simulink model "PMLSM_ControlCore_Block"  (R2026a)
settings: Solver=FixedStepDiscrete  StopTime=1  FixedStep=1e-4
values from neighbouring files (symbols this model uses):
  CPU_Clock = 200e6    (= 200000000)    [PMSLM_Init_Params_MBDL4.m]
  Current_Control_Mode = 2    [init_PMLSM_mil_test_params.m]
  DeadTime_Comp_Enable = 0    [init_PMLSM_mil_test_params.m]
  delay_N = 50    [PMSLM_Init_Params_MBDL4.m]
  DPCC_Ld_Factor = 1    [init_PMLSM_mil_test_params.m]
  DPCC_Lq_Factor = 1    [init_PMLSM_mil_test_params.m]
  DPCC_Psi_Factor = 1    [init_PMLSM_mil_test_params.m]
  DPCC_Rs_Factor = 1    [init_PMLSM_mil_test_params.m]
  DPICC_Ld_Factor = 1    [init_PMLSM_mil_test_params.m]
  DPICC_Lq_Factor = 1    [init_PMLSM_mil_test_params.m]
  Hold_Ticks = 30000    [PMSLM_Init_Params_MBDL4.m]
  Id_Init_Step = Id_Init_Target / Ramp_Ticks    (= 5e-05)    [PMSLM_Init_Params_MBDL4.m]
  Id_Init_Target = 0.5    [PMSLM_Init_Params_MBDL4.m]
  Id_Release_Ramp_Ticks = 2000    [PMSLM_Init_Params_MBDL4.m]
  Iq_fric_run = 0.05    [PMSLM_Init_Params_MBDL4.m]
  Iq_fric_start = 0.40    (= 0.4)    [PMSLM_Init_Params_MBDL4.m]
  Iq_int_limit = 0.10    (= 0.1)    [PMSLM_Init_Params_MBDL4.m]
  Kaw_d = Kaw_q    (= 0.2)    [PMSLM_Init_Params_MBDL4.m]
  Kaw_q = 0.2    [PMSLM_Init_Params_MBDL4.m]
  Kaw_s = 0.4    [PMSLM_Init_Params_MBDL4.m]
  Ki_ACR = ACR_Commissioning_Scale*Ki_ACR_Baseline    (= 2962.5)    [PMSLM_Init_Params_MBDL4.m]    (also in init_PMLSM_mil_test_params.m = Kp_ACR*PMLSM_Rs_ohm/PMLSM_Lq_H)
  Ki_ASR = 0.05    [PMSLM_Init_Params_MBDL4.m]
  Kp_ACR = ACR_Commissioning_Scale*Kp_ACR_Baseline    (= 2.18125)    [PMSLM_Init_Params_MBDL4.m]    (also in init_PMLSM_mil_test_params.m = PMLSM_Lq_H/(4*MIL_AUM3S4_Current_PI_xi^2*MIL_AUM3S4_Current_)
  Kp_ASR = 0.03    [PMSLM_Init_Params_MBDL4.m]
  Kp_pos = 5    [PMSLM_Init_Params_MBDL4.m]
  PICDO_Dhat_Limit_A = 3.0    (= 3)    [init_PMLSM_mil_test_params.m]
  PICDO_Kd = 0.25    [init_PMLSM_mil_test_params.m]
  PICDO_Kx = 1.0    (= 1)    [init_PMLSM_mil_test_params.m]
  PMLSM_deadtime_ratio = PMLSM_deadtime_s * PMLSM_pwm_freq_Hz    (= 0.01)    [init_PMLSM_plant_params.m]
  PMLSM_Ld_H = Ld    (= 0.001745)    [PMSLM_Init_Params_MBDL4.m]    (also in init_PMLSM_plant_params.m)
  PMLSM_Lq_H = Lq    (= 0.001745)    [PMSLM_Init_Params_MBDL4.m]    (also in init_PMLSM_plant_params.m)
  PMLSM_psi_f_Wb = flux    (= 0.141)    [PMSLM_Init_Params_MBDL4.m]    (also in init_PMLSM_plant_params.m)
  PMLSM_Rs_ohm = Rs    (= 2.37)    [PMSLM_Init_Params_MBDL4.m]    (also in init_PMLSM_plant_params.m)
  Pos_deadband = 0.02    [PMSLM_Init_Params_MBDL4.m]
  Ramp_Ticks = 10000    [PMSLM_Init_Params_MBDL4.m]
  Speed_Feedback_Mode = 1    [init_PMLSM_mil_test_params.m]
  Speed_loop_Iq_Limit = Iq_Limit    (= 0.3)    [PMSLM_Init_Params_MBDL4.m]
  Tau_e_mm = 60    [PMSLM_Init_Params_MBDL4.m]
  theta_align_const = 0    [PMSLM_Init_Params_MBDL4.m]
  Theta_Offset_Fine = Simulink.Parameter    [PMSLM_Init_Params_MBDL4.m]
  Ts = 1 / PWM_Freq    (= 0.0001)    [PMSLM_Init_Params_MBDL4.m]
  Ts_ACR = 1e-4    (= 0.0001)    [PMSLM_Init_Params_MBDL4.m]
  Ts_ASR = 1e-3    (= 0.001)    [PMSLM_Init_Params_MBDL4.m]
  Ts_DPICC = 1e-4    (= 0.0001)    [init_PMLSM_mil_test_params.m]
  Udc = 48    [PMSLM_Init_Params_MBDL4.m]    (also in init_PMLSM_mil_test_params.m)
  Uq_Zero_EN = 0：q 轴用正常 PI    [PMSLM_Init_Params_MBDL4.m]
  v_ff_eps = 0.5    [PMSLM_Init_Params_MBDL4.m]
  V_meas_max = 500    [PMSLM_Init_Params_MBDL4.m]
  v_meas_zero_eps = 0.5    [PMSLM_Init_Params_MBDL4.m]
  v_over_eps = 3    [PMSLM_Init_Params_MBDL4.m]
  V_pos_max_mmps = 10    [PMSLM_Init_Params_MBDL4.m]
  v_ref_max = 20    [PMSLM_Init_Params_MBDL4.m]
  v_ref_set_step_dn = v_ref_set_rate_dn * Ts    (= 0.005)    [PMSLM_Init_Params_MBDL4.m]
  v_ref_set_step_up = v_ref_set_rate_up * Ts    (= 0.005)    [PMSLM_Init_Params_MBDL4.m]
  v_ref_zero_eps = 0.2    [PMSLM_Init_Params_MBDL4.m]
  v_stick_off = 3.0    (= 3)    [PMSLM_Init_Params_MBDL4.m]
  v_stick_on = 1.0    (= 1)    [PMSLM_Init_Params_MBDL4.m]
  X_max_hard = 500    [PMSLM_Init_Params_MBDL4.m]
  X_max_soft = 470    [PMSLM_Init_Params_MBDL4.m]
  X_min_hard = -500    [PMSLM_Init_Params_MBDL4.m]
  X_min_soft = -470    [PMSLM_Init_Params_MBDL4.m]
libraries: hdlsllib x13, simulink x11, mcbeeMathTransformLib x2, mcbcontrolslib x1
(part 1 of 3)
settings Model: Creator=lww  LastModifiedBy=lww
settings ModelReferenceCC: ModelReferenceNumInstancesAllowed=Single
settings GRTTargetCC: SubcomponentCodeInterfacePackaging=Nonreusable function

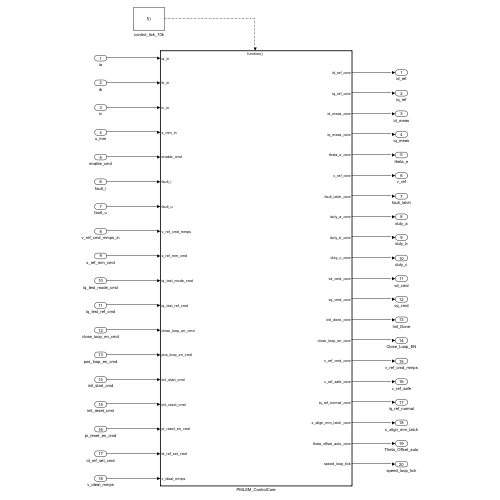
[thumbnail: Simulink's stored preview of the top-level diagram]
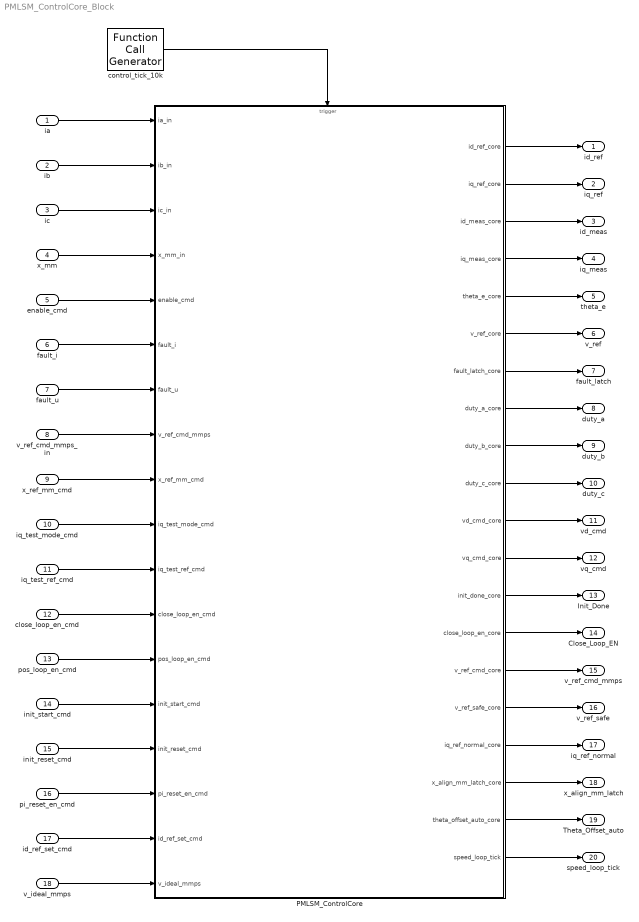
== system PMLSM_ControlCore_Block ==
  ia : Inport
  ib : Inport  Port=2
  ic : Inport  Port=3
  x_mm : Inport  Port=4
  enable_cmd : Inport  Port=5
  fault_i : Inport  Port=6
  fault_u : Inport  Port=7
  v_ref_cmd_mmps_in : Inport  Port=8
  x_ref_mm_cmd : Inport  Port=9
  iq_test_mode_cmd : Inport  Port=10
  iq_test_ref_cmd : Inport  Port=11
  close_loop_en_cmd : Inport  Port=12
  pos_loop_en_cmd : Inport  Port=13
  init_start_cmd : Inport  Port=14
  init_reset_cmd : Inport  Port=15
  pi_reset_en_cmd : Inport  Port=16
  id_ref_set_cmd : Inport  Port=17
  v_ideal_mmps : Inport  Port=18
  PMLSM_ControlCore : Subsystem  TreatAsAtomicUnit=on
  control_tick_10k : FunctionCallGenerator  SampleTime=1e-4
  id_ref : Outport
  iq_ref : Outport  Port=2
  id_meas : Outport  Port=3
  iq_meas : Outport  Port=4
  theta_e : Outport  Port=5
  v_ref : Outport  Port=6
  fault_latch : Outport  Port=7
  duty_a : Outport  Port=8
  duty_b : Outport  Port=9
  duty_c : Outport  Port=10
  vd_cmd : Outport  Port=11
  vq_cmd : Outport  Port=12
  Init_Done : Outport  Port=13
  Close_Loop_EN : Outport  Port=14
  v_ref_cmd_mmps : Outport  Port=15
  v_ref_safe : Outport  Port=16
  iq_ref_normal : Outport  Port=17
  x_align_mm_latch : Outport  Port=18
  Theta_Offset_auto : Outport  Port=19
  speed_loop_tick : Outport  Port=20
  wires:
  ia/1 -> PMLSM_ControlCore/1(ia_in)
  ib/1 -> PMLSM_ControlCore/2(ib_in)
  ic/1 -> PMLSM_ControlCore/3(ic_in)
  x_mm/1 -> PMLSM_ControlCore/4(x_mm_in)
  enable_cmd/1 -> PMLSM_ControlCore/5(enable_cmd)
  fault_i/1 -> PMLSM_ControlCore/6(fault_i)
  fault_u/1 -> PMLSM_ControlCore/7(fault_u)
  v_ref_cmd_mmps_in/1 -> PMLSM_ControlCore/8(v_ref_cmd_mmps)
  x_ref_mm_cmd/1 -> PMLSM_ControlCore/9(x_ref_mm_cmd)
  iq_test_mode_cmd/1 -> PMLSM_ControlCore/10(iq_test_mode_cmd)
  iq_test_ref_cmd/1 -> PMLSM_ControlCore/11(iq_test_ref_cmd)
  close_loop_en_cmd/1 -> PMLSM_ControlCore/12(close_loop_en_cmd)
  pos_loop_en_cmd/1 -> PMLSM_ControlCore/13(pos_loop_en_cmd)
  init_start_cmd/1 -> PMLSM_ControlCore/14(init_start_cmd)
  init_reset_cmd/1 -> PMLSM_ControlCore/15(init_reset_cmd)
  pi_reset_en_cmd/1 -> PMLSM_ControlCore/16(pi_reset_en_cmd)
  id_ref_set_cmd/1 -> PMLSM_ControlCore/17(id_ref_set_cmd)
  control_tick_10k/1 -> PMLSM_ControlCore/Trigger
  PMLSM_ControlCore/1(id_ref_core) -> id_ref/1
  PMLSM_ControlCore/2(iq_ref_core) -> iq_ref/1
  PMLSM_ControlCore/3(id_meas_core) -> id_meas/1
  PMLSM_ControlCore/4(iq_meas_core) -> iq_meas/1
  PMLSM_ControlCore/5(theta_e_core) -> theta_e/1
  PMLSM_ControlCore/6(v_ref_core) -> v_ref/1
  PMLSM_ControlCore/7(fault_latch_core) -> fault_latch/1
  PMLSM_ControlCore/8(duty_a_core) -> duty_a/1
  PMLSM_ControlCore/9(duty_b_core) -> duty_b/1
  PMLSM_ControlCore/10(duty_c_core) -> duty_c/1
  PMLSM_ControlCore/11(vd_cmd_core) -> vd_cmd/1
  PMLSM_ControlCore/12(vq_cmd_core) -> vq_cmd/1
  PMLSM_ControlCore/13(init_done_core) -> Init_Done/1
  PMLSM_ControlCore/14(close_loop_en_core) -> Close_Loop_EN/1
  PMLSM_ControlCore/15(v_ref_cmd_core) -> v_ref_cmd_mmps/1
  PMLSM_ControlCore/16(v_ref_safe_core) -> v_ref_safe/1
  PMLSM_ControlCore/17(iq_ref_normal_core) -> iq_ref_normal/1
  PMLSM_ControlCore/18(x_align_mm_latch_core) -> x_align_mm_latch/1
  PMLSM_ControlCore/19(theta_offset_auto_core) -> Theta_Offset_auto/1
  v_ideal_mmps/1 -> PMLSM_ControlCore/18(v_ideal_mmps)
  PMLSM_ControlCore/20(speed_loop_tick) -> speed_loop_tick/1

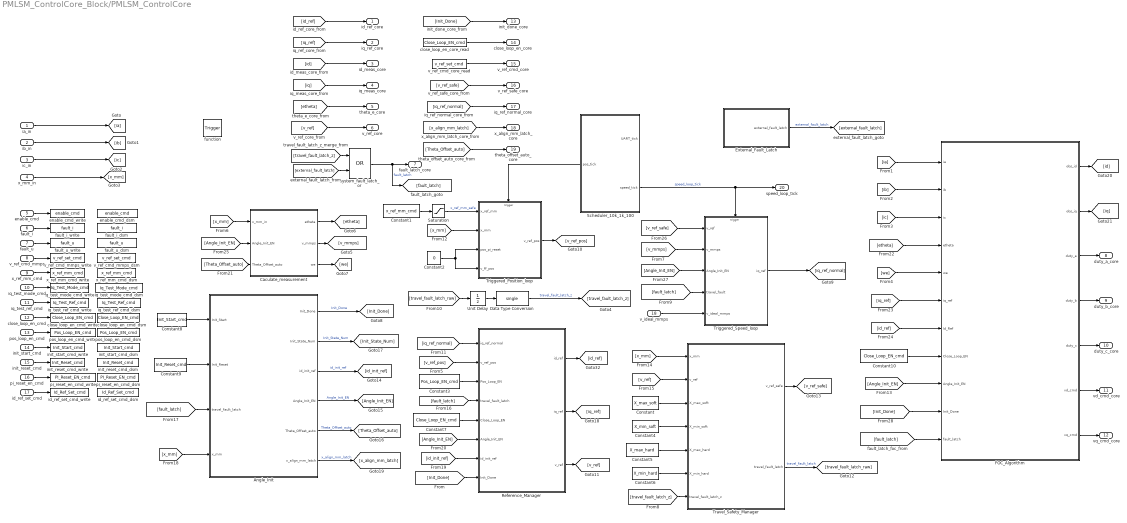
== system PMLSM_ControlCore_Block/PMLSM_ControlCore ==
  ia_in : Inport
  ib_in : Inport  Port=2
  ic_in : Inport  Port=3
  x_mm_in : Inport  Port=4
  enable_cmd : Inport  Port=5
  fault_i : Inport  Port=6
  fault_u : Inport  Port=7
  v_ref_cmd_mmps : Inport  Port=8
  x_ref_mm_cmd : Inport  Port=9
  iq_test_mode_cmd : Inport  Port=10
  iq_test_ref_cmd : Inport  Port=11
  close_loop_en_cmd : Inport  Port=12
  pos_loop_en_cmd : Inport  Port=13
  init_start_cmd : Inport  Port=14
  init_reset_cmd : Inport  Port=15
  pi_reset_en_cmd : Inport  Port=16
  id_ref_set_cmd : Inport  Port=17
  v_ideal_mmps : Inport  Port=18
  function : TriggerPort  TriggerType=function-call  VariantControl=(inherit)
  Angle_Init : Stateflow chart  TreatAsAtomicUnit=on
  Caculate_measurement : Subsystem
  Constant : Constant  Value=X_max_soft
  Constant1 : DataStoreRead  DataStoreName=x_ref_mm_cmd  IndexOptions=Index vector (dialog)  Indices=1  OutputSizes=1
  Constant10 : DataStoreRead  DataStoreName=Close_Loop_EN_cmd  IndexOptions=Index vector (dialog)  Indices=1  OutputSizes=1
  Constant2 : Constant  Value=0
  Constant3 : DataStoreRead  DataStoreName=Pos_Loop_EN_cmd  IndexOptions=Index vector (dialog)  Indices=1  OutputSizes=1
  Constant4 : Constant  Value=X_min_soft
  Constant5 : Constant  Value=X_max_hard
  Constant6 : Constant  Value=X_min_hard
  Constant7 : DataStoreRead  DataStoreName=Close_Loop_EN_cmd  IndexOptions=Index vector (dialog)  Indices=1  OutputSizes=1
  Constant8 : DataStoreRead  DataStoreName=Init_Start_cmd  IndexOptions=Index vector (dialog)  Indices=1  OutputSizes=1
  Constant9 : DataStoreRead  DataStoreName=Init_Reset_cmd  IndexOptions=Index vector (dialog)  Indices=1  OutputSizes=1
  Data Type Conversion : DataTypeConversion  OutDataTypeStr=single  SaturateOnIntegerOverflow=off  RndMeth=Floor
  External_Fault_Latch : Subsystem
  FOC_Algorithm : Subsystem
  Reference_Manager : Subsystem
  Saturation : Saturate  UpperLimit=X_max_soft  LowerLimit=X_min_soft
  Scheduler_10k_1k_100 : Subsystem
      settings: PortSchema="{\"entries\":[{\"content\":{\"sides\":[{\"content\":{\"connectorIds\":[\"Out3\"]},\"type\":\"ConnectorPlacement.EquallySpacedRectSide\",\"uuid\":\"7a2cd2ad-1b6d-4ced-b4c0-dea2e76e4441\"},{\"content\":{\"connectorIds\":[\"Out1\",\"Out2\"],\"side\":\"RIGHT\"},\"type\":\"ConnectorPlacement.EquallySpacedRectSide\",\"uuid\":\"f7db3b94-1126-4089-83bd-8e57d20e6fd7\"},{\"content\":{\"side\":\"TOP\"},\"type\":\"ConnectorPlacement.EquallySpacedRectSide\",\"uuid\":\"9153f6b5-22af-48be-92c0-68be43f93648\"}]},\"type\":\"ConnectorPlacement.EquallySpacedConnector\",\"uuid\":\"029fb485-bddc-4cd2-9c64-7547c8dffd2b\"}],\"packageUris\":[\"http://schema.mathworks.com/mf0/Connector/R2020b\"],\"version\":\"1.0\"}"
  Travel_Safety_Manager : MATLAB Function  TreatAsAtomicUnit=on
  Triggered_Position_loop : Subsystem  TreatAsAtomicUnit=on
  Triggered_Speed_loop : Subsystem  TreatAsAtomicUnit=on
  Unit Delay : UnitDelay  SampleTime=-1
  close_loop_en_cmd_dsm : DataStoreMemory  DataStoreName=Close_Loop_EN_cmd  ShowAdditionalParam=off
  close_loop_en_cmd_write : DataStoreWrite  DataStoreName=Close_Loop_EN_cmd  IndexOptions=Index vector (dialog)  Indices=1  OutputSizes=1
  close_loop_en_core_read : DataStoreRead  DataStoreName=Close_Loop_EN_cmd  IndexOptions=Index vector (dialog)  Indices=1  OutputSizes=1
  enable_cmd_dsm : DataStoreMemory  DataStoreName=enable_cmd  ShowAdditionalParam=off
  enable_cmd_write : DataStoreWrite  DataStoreName=enable_cmd  IndexOptions=Index vector (dialog)  Indices=1  OutputSizes=1
  fault_i_dsm : DataStoreMemory  DataStoreName=fault_i  ShowAdditionalParam=off
  fault_i_write : DataStoreWrite  DataStoreName=fault_i  IndexOptions=Index vector (dialog)  Indices=1  OutputSizes=1
  fault_u_dsm : DataStoreMemory  DataStoreName=fault_u  ShowAdditionalParam=off
  fault_u_write : DataStoreWrite  DataStoreName=fault_u  IndexOptions=Index vector (dialog)  Indices=1  OutputSizes=1
  id_ref_set_cmd_dsm : DataStoreMemory  DataStoreName=Id_Ref_Set_cmd  ShowAdditionalParam=off
  id_ref_set_cmd_write : DataStoreWrite  DataStoreName=Id_Ref_Set_cmd  IndexOptions=Index vector (dialog)  Indices=1  OutputSizes=1
  init_reset_cmd_dsm : DataStoreMemory  DataStoreName=Init_Reset_cmd  ShowAdditionalParam=off
  init_reset_cmd_write : DataStoreWrite  DataStoreName=Init_Reset_cmd  IndexOptions=Index vector (dialog)  Indices=1  OutputSizes=1
  init_start_cmd_dsm : DataStoreMemory  DataStoreName=Init_Start_cmd  ShowAdditionalParam=off
  init_start_cmd_write : DataStoreWrite  DataStoreName=Init_Start_cmd  IndexOptions=Index vector (dialog)  Indices=1  OutputSizes=1
  iq_test_mode_cmd_dsm : DataStoreMemory  DataStoreName=Iq_Test_Mode_cmd  ShowAdditionalParam=off
  iq_test_mode_cmd_write : DataStoreWrite  DataStoreName=Iq_Test_Mode_cmd  IndexOptions=Index vector (dialog)  Indices=1  OutputSizes=1
  iq_test_ref_cmd_dsm : DataStoreMemory  DataStoreName=Iq_Test_Ref_cmd  ShowAdditionalParam=off
  iq_test_ref_cmd_write : DataStoreWrite  DataStoreName=Iq_Test_Ref_cmd  IndexOptions=Index vector (dialog)  Indices=1  OutputSizes=1
  pi_reset_en_cmd_dsm : DataStoreMemory  DataStoreName=PI_Reset_EN_cmd  ShowAdditionalParam=off
  pi_reset_en_cmd_write : DataStoreWrite  DataStoreName=PI_Reset_EN_cmd  IndexOptions=Index vector (dialog)  Indices=1  OutputSizes=1
  pos_loop_en_cmd_dsm : DataStoreMemory  DataStoreName=Pos_Loop_EN_cmd  ShowAdditionalParam=off
  pos_loop_en_cmd_write : DataStoreWrite  DataStoreName=Pos_Loop_EN_cmd  IndexOptions=Index vector (dialog)  Indices=1  OutputSizes=1
  system_fault_latch_or : Logic  Operator=OR  AllPortsSameDT=off  OutDataTypeStr=boolean
  v_ref_cmd_core_read : DataStoreRead  DataStoreName=v_ref_set_cmd  IndexOptions=Index vector (dialog)  Indices=1  OutputSizes=1
  v_ref_cmd_mmps_dsm : DataStoreMemory  DataStoreName=v_ref_set_cmd  ShowAdditionalParam=off
  v_ref_cmd_mmps_write : DataStoreWrite  DataStoreName=v_ref_set_cmd  IndexOptions=Index vector (dialog)  Indices=1  OutputSizes=1
  x_ref_mm_cmd_dsm : DataStoreMemory  DataStoreName=x_ref_mm_cmd  ShowAdditionalParam=off
  x_ref_mm_cmd_write : DataStoreWrite  DataStoreName=x_ref_mm_cmd  IndexOptions=Index vector (dialog)  Indices=1  OutputSizes=1
  id_ref_core : Outport
  iq_ref_core : Outport  Port=2
  id_meas_core : Outport  Port=3
  iq_meas_core : Outport  Port=4
  theta_e_core : Outport  Port=5
  v_ref_core : Outport  Port=6
  fault_latch_core : Outport  Port=7
  duty_a_core : Outport  Port=8
  duty_b_core : Outport  Port=9
  duty_c_core : Outport  Port=10
  vd_cmd_core : Outport  Port=11
  vq_cmd_core : Outport  Port=12
  init_done_core : Outport  Port=13
  close_loop_en_core : Outport  Port=14
  v_ref_cmd_core : Outport  Port=15
  v_ref_safe_core : Outport  Port=16
  iq_ref_normal_core : Outport  Port=17
  x_align_mm_latch_core : Outport  Port=18
  theta_offset_auto_core : Outport  Port=19
  speed_loop_tick : Outport  Port=20
  wires:
  Scheduler_10k_1k_100/3(pos_tick) -> Triggered_Position_loop/Trigger
  FOC_Algorithm/2(obs_iq) -> [iq]
  FOC_Algorithm/1(obs_id) -> [id]
  Angle_Init/6(x_align_mm_latch) -> [x_align_mm_latch]  "x_align_mm_latch"
  [Angle_Init_EN] -> Triggered_Speed_loop/3(Angle_Init_EN)
  Angle_Init/2(Init_State_Num) -> [Init_State_Num]  "Init_State_Num"
  [Angle_Init_EN] -> Caculate_measurement/2(Angle_Init_EN)
  [Theta_Offset_auto] -> Caculate_measurement/3(Theta_Offset_auto)
  Angle_Init/5(Theta_Offset_auto) -> [Theta_Offset_auto]  "Theta_Offset_auto"
  [Angle_Init_EN] -> Reference_Manager/6(Angle_Init_EN)
  Angle_Init/4(Angle_Init_EN) -> [Angle_Init_EN]  "Angle_Init_EN"
  [id_init_ref] -> Reference_Manager/7(id_init_ref)
  Angle_Init/3(id_init_ref) -> [id_init_ref]  "id_init_ref"
  [x_mm] -> Angle_Init/4(x_mm)
  [Init_Done] -> Reference_Manager/8(Init_Done)
  Angle_Init/1(Init_Done) -> [Init_Done]  "Init_Done"
  [fault_latch] -> Angle_Init/3(travel_fault_latch)
  [fault_latch] -> Reference_Manager/4(travel_fault_latch)
  Data Type Conversion/1 -> [travel_fault_latch_z]  "travel_fault_latch_z"
  Unit Delay/1 -> Data Type Conversion/1
  [travel_fault_latch_z] -> Travel_Safety_Manager/7(travel_fault_latch_z)
  Travel_Safety_Manager/1(v_ref_safe) -> [v_ref_safe]
  Travel_Safety_Manager/2(travel_fault_latch) -> [travel_fault_latch_raw]  "travel_fault_latch"
  Constant6/1 -> Travel_Safety_Manager/6(X_min_hard)
  Constant5/1 -> Travel_Safety_Manager/5(X_max_hard)
  Constant4/1 -> Travel_Safety_Manager/4(X_min_soft)
  Constant/1 -> Travel_Safety_Manager/3(X_max_soft)
  [v_ref] -> Travel_Safety_Manager/2(v_ref)
  [x_mm] -> Travel_Safety_Manager/1(x_mm)
  [id_ref] -> FOC_Algorithm/7(Id_Ref)
  [travel_fault_latch_raw] -> Unit Delay/1
  [fault_latch] -> Triggered_Speed_loop/4(travel_fault)
  Saturation/1 -> Triggered_Position_loop/1(x_ref_mm)  "x_ref_mm_safe"
  Reference_Manager/3(v_ref) -> [v_ref]
  [x_mm] -> Caculate_measurement/1(x_mm_in)
  Caculate_measurement/3(we) -> [we]
  [v_ref_pos] -> Reference_Manager/2(v_ref_pos)
  Triggered_Position_loop/1(v_ref_pos) -> [v_ref_pos]
  Constant2/1 -> Triggered_Position_loop/3(pos_pi_reset), Triggered_Position_loop/4(v_ff_pos)
  [x_mm] -> Triggered_Position_loop/2(x_mm)
  [iq_ref] -> FOC_Algorithm/6(iq_ref)
  [we] -> FOC_Algorithm/5(we)
  [etheta] -> FOC_Algorithm/4(etheta)
  [ic] -> FOC_Algorithm/3(ic)
  [ib] -> FOC_Algorithm/2(ib)
  [ia] -> FOC_Algorithm/1(ia)
  Triggered_Speed_loop/1(iq_ref) -> [iq_ref_normal]
  Reference_Manager/2(iq_ref) -> [iq_ref]
  [v_ref_safe] -> Triggered_Speed_loop/1(v_ref)
  Scheduler_10k_1k_100/2(speed_tick) -> speed_loop_tick/1, Triggered_Speed_loop/Trigger  "speed_loop_tick"
  Reference_Manager/1(id_ref) -> [id_ref]
  Caculate_measurement/1(etheta) -> [etheta]
  [v_mmps] -> Triggered_Speed_loop/2(v_mmps)
  Caculate_measurement/2(v_mmps) -> [v_mmps]
  [iq_ref_normal] -> Reference_Manager/1(iq_ref_normal)
  ia_in/1 -> [ia]
  ib_in/1 -> [ib]
  ic_in/1 -> [ic]
  x_mm_in/1 -> [x_mm]
  enable_cmd/1 -> enable_cmd_write/1
  fault_i/1 -> fault_i_write/1
  fault_u/1 -> fault_u_write/1
  v_ref_cmd_mmps/1 -> v_ref_cmd_mmps_write/1
  x_ref_mm_cmd/1 -> x_ref_mm_cmd_write/1
  Constant1/1 -> Saturation/1
  iq_test_mode_cmd/1 -> iq_test_mode_cmd_write/1
  iq_test_ref_cmd/1 -> iq_test_ref_cmd_write/1
  close_loop_en_cmd/1 -> close_loop_en_cmd_write/1
  Constant7/1 -> Reference_Manager/5(Close_Loop_EN)
  pos_loop_en_cmd/1 -> pos_loop_en_cmd_write/1
  Constant3/1 -> Reference_Manager/3(Pos_Loop_EN)
  init_start_cmd/1 -> init_start_cmd_write/1
  Constant8/1 -> Angle_Init/1(Init_Start)
  init_reset_cmd/1 -> init_reset_cmd_write/1
  Constant9/1 -> Angle_Init/2(Init_Reset)
  pi_reset_en_cmd/1 -> pi_reset_en_cmd_write/1
  id_ref_set_cmd/1 -> id_ref_set_cmd_write/1
  [id_ref] -> id_ref_core/1
  [iq_ref] -> iq_ref_core/1
  [id] -> id_meas_core/1
  [iq] -> iq_meas_core/1
  [etheta] -> theta_e_core/1
  [v_ref] -> v_ref_core/1
  [Init_Done] -> init_done_core/1
  close_loop_en_core_read/1 -> close_loop_en_core/1
  v_ref_cmd_core_read/1 -> v_ref_cmd_core/1
  [v_ref_safe] -> v_ref_safe_core/1
  [iq_ref_normal] -> iq_ref_normal_core/1
  [x_align_mm_latch] -> x_align_mm_latch_core/1
  [Theta_Offset_auto] -> theta_offset_auto_core/1
  [travel_fault_latch_z] -> system_fault_latch_or/1
  External_Fault_Latch/1(external_fault_latch) -> [external_fault_latch]  "external_fault_latch"
  [external_fault_latch] -> system_fault_latch_or/2
  system_fault_latch_or/1 -> fault_latch_core/1, [fault_latch]  "fault_latch"
  FOC_Algorithm/3(duty_a) -> duty_a_core/1
  FOC_Algorithm/4(duty_b) -> duty_b_core/1
  FOC_Algorithm/5(duty_c) -> duty_c_core/1
  FOC_Algorithm/6(vd_cmd) -> vd_cmd_core/1
  FOC_Algorithm/7(vq_cmd) -> vq_cmd_core/1
  v_ideal_mmps/1 -> Triggered_Speed_loop/5(v_ideal_mmps)
  [Angle_Init_EN] -> FOC_Algorithm/9(Angle_Init_EN)
  Constant10/1 -> FOC_Algorithm/8(Close_Loop_EN)
  [fault_latch] -> FOC_Algorithm/11(fault_latch)
  [Init_Done] -> FOC_Algorithm/10(Init_Done)

== system PMLSM_ControlCore_Block/PMLSM_ControlCore/Caculate_measurement ==
  x_mm_in : Inport
  Angle_Init_EN : Inport  Port=2
  Theta_Offset_auto : Inport  Port=3
  Add1 : Sum  Inputs=+-
  Add2 : Sum  Inputs=+++
  Constant : Constant  Value=0
  Constant1 : Constant  Value=0
  Constant4 : Constant  Value=2*pi
  Constant6 : Constant  Value=theta_align_const
  Data Type Conversion : DataTypeConversion  OutDataTypeStr=double  SaturateOnIntegerOverflow=off  RndMeth=Floor
  Delay : Delay  DelayLength=50
  Gain : Gain  Gain=2*pi/Tau_e_mm
  Gain1 : Gain  Gain=1/(delay_N*Ts)
  Gain2 : Gain  Gain=2*pi/Tau_e_mm
  IIR Filter : Subsystem  TreatAsAtomicUnit=on
  Math Function1 : Math  Operator=mod
  Saturation : Saturate  UpperLimit=V_meas_max  LowerLimit=-V_meas_max
  Switch : Switch  Criteria=u2 > Threshold  Threshold=0.5  SaturateOnIntegerOverflow=off  InputSameDT=off
  Switch1 : Switch  Criteria=u2 > Threshold  Threshold=0.5  SaturateOnIntegerOverflow=off  InputSameDT=off
  Switch2 : Switch  Criteria=u2 > Threshold  Threshold=0.5  SaturateOnIntegerOverflow=off  InputSameDT=off
  Theta_Offset : Constant  Value=Theta_Offset_Fine
  etheta : Outport
  v_mmps : Outport  Port=2
  we : Outport  Port=3
  wires:
  Theta_Offset_auto/1 -> Add2/2
  Theta_Offset/1 -> Add2/3
  [Angle_Init_EN] -> IIR Filter/Reset, Switch1/2
  Gain2/1 -> we/1
  Constant6/1 -> Switch2/1
  Angle_Init_EN/1 -> [Angle_Init_EN]
  Switch2/1 -> etheta/1  "obs_etheta"
  Math Function1/1 -> Switch2/3  "theta_calc"
  [Angle_Init_EN] -> Switch2/2, Switch/2
  Saturation/1 -> Switch/3
  Gain1/1 -> IIR Filter/1(In1)
  IIR Filter/1(Out1) -> Saturation/1
  Add1/1 -> Switch1/3
  Switch1/1 -> Gain1/1
  Constant1/1 -> Switch1/1
  Constant/1 -> Switch/1
  Switch/1 -> v_mmps/1, Gain2/1  "obs_v_mmps"
  Data Type Conversion/1 -> Gain/1, Add1/1, Delay/1
  Constant4/1 -> Math Function1/2
  Add2/1 -> Math Function1/1
  Gain/1 -> Add2/1
  Delay/1 -> Add1/2  "x_mm_delay"
  x_mm_in/1 -> Data Type Conversion/1

== system PMLSM_ControlCore_Block/PMLSM_ControlCore/External_Fault_Latch ==
  external_fault_latch_or : Logic  Operator=OR  AllPortsSameDT=off  OutDataTypeStr=boolean
  external_fault_latch_z : UnitDelay  SampleTime=-1
  external_fault_or : Logic  Operator=OR  AllPortsSameDT=off  OutDataTypeStr=boolean
  fault_i : DataStoreRead  DataStoreName=fault_i  IndexOptions=Index vector (dialog)  Indices=1  OutputSizes=1
  fault_i_active : simulink/Logic and Bit Operations/Compare To Constant  relop=~=  const=0  OutDataTypeStr=boolean
  fault_u : DataStoreRead  DataStoreName=fault_u  IndexOptions=Index vector (dialog)  Indices=1  OutputSizes=1
  fault_u_active : simulink/Logic and Bit Operations/Compare To Constant  relop=~=  const=0  OutDataTypeStr=boolean
  external_fault_latch : Outport
  wires:
  fault_i/1 -> fault_i_active/1
  fault_u/1 -> fault_u_active/1
  fault_i_active/1 -> external_fault_or/1
  fault_u_active/1 -> external_fault_or/2
  external_fault_or/1 -> external_fault_latch_or/1
  external_fault_latch_z/1 -> external_fault_latch_or/2
  external_fault_latch_or/1 -> external_fault_latch_z/1, external_fault_latch/1

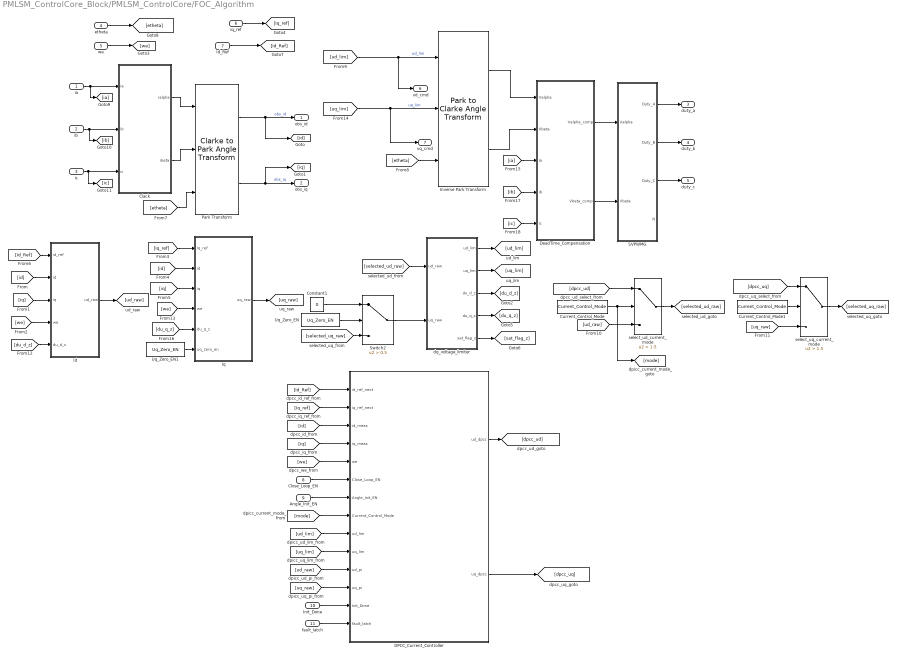
== system PMLSM_ControlCore_Block/PMLSM_ControlCore/FOC_Algorithm ==
  ia : Inport
  ib : Inport  Port=2
  ic : Inport  Port=3
  etheta : Inport  Port=4
  we : Inport  Port=5
  iq_ref : Inport  Port=6
  Id_Ref : Inport  Port=7
  Close_Loop_EN : Inport  Port=8
  Angle_Init_EN : Inport  Port=9
  Init_Done : Inport  Port=10
  fault_latch : Inport  Port=11
  Clack : Subsystem  TreatAsAtomicUnit=on  RTWFcnName=Clack_Fun
      settings: RTWFcnNameOpts=User specified
  Constant1 : Constant  Value=0  OutDataTypeStr=double
  Current_Control_Mode : Constant  Value=Current_Control_Mode
  Current_Control_Mode1 : Constant  Value=Current_Control_Mode
  DPCC_Current_Controller : Subsystem
  DeadTime_Compensation : Subsystem
  Id : Subsystem  TreatAsAtomicUnit=on  RTWFcnName=Id_Fun
      settings: RTWFcnNameOpts=User specified
  Inverse Park Transform : mcbeeMathTransformLib/Park to Clarke Angle Transform  AxisAlignment=D-axis  UseWithEmbedded=on  PhaseInput=Two inputs  ThetaInput=Electrical position  AngleInput=Radians  N_points=1024
      settings: LibrarySourceBlock=mcbhdllib/Controls/Math Transforms/Inverse Park Transform
  Iq : Subsystem  TreatAsAtomicUnit=on  RTWFcnName=Iq_Fun
      settings: RTWFcnNameOpts=User specified
  Park Transform : mcbeeMathTransformLib/Clarke to Park Angle Transform  AxisAlignment=D-axis  UseWithEmbedded=on  PhaseInput=Two inputs  ThetaInput=Electrical position  AngleInput=Radians  N_points=1024
      settings: LibrarySourceBlock=mcblib/Controls/Math Transforms/Park Transform
  SVPWMG : Subsystem  TreatAsAtomicUnit=on  RTWFcnName=SVPWM_Gen_Fun
      settings: RTWFcnNameOpts=User specified
  Switch2 : Switch  Criteria=u2 > Threshold  Threshold=0.5  SaturateOnIntegerOverflow=off  InputSameDT=off
  Uq_Zero_EN : Constant  Value=Uq_Zero_EN
  Uq_Zero_EN1 : Constant  Value=Uq_Zero_EN
  dq_voltage_limiter : Subsystem
  select_ud_current_mode : Switch  Criteria=u2 > Threshold  Threshold=1.5  SaturateOnIntegerOverflow=off  InputSameDT=off
  select_uq_current_mode : Switch  Criteria=u2 > Threshold  Threshold=1.5  SaturateOnIntegerOverflow=off  InputSameDT=off
  obs_id : Outport
  obs_iq : Outport  Port=2
  duty_a : Outport  Port=3
  duty_b : Outport  Port=4
  duty_c : Outport  Port=5
  vd_cmd : Outport  Port=6
  vq_cmd : Outport  Port=7
  wires:
  Clack/1(ialpha) -> Park Transform/1
  Clack/2(ibeta) -> Park Transform/2
  Uq_Zero_EN1/1 -> Iq/6(uq_zero_en)
  we/1 -> [we]
  [etheta] -> Inverse Park Transform/3
  etheta/1 -> [etheta]
  Id_Ref/1 -> [Id_Ref]
  [Id_Ref] -> Id/1(id_ref)
  dq_voltage_limiter/5(sat_flag_z) -> [sat_flag_z]
  [Iq_ref] -> Iq/1(Iq_ref)
  Switch2/1 -> dq_voltage_limiter/2(uq_raw)
  Constant1/1 -> Switch2/1
  Uq_Zero_EN/1 -> Switch2/2
  [du_q_z] -> Iq/5(du_q_z)
  [du_d_z] -> Id/5(du_d_z)
  dq_voltage_limiter/4(du_q_z) -> [du_q_z]
  dq_voltage_limiter/3(du_d_z) -> [du_d_z]
  dq_voltage_limiter/2(uq_lim) -> [uq_lim]
  dq_voltage_limiter/1(ud_lim) -> [ud_lim]
  Iq/1(uq_raw) -> [uq_raw]
  Id/1(ud_raw) -> [ud_raw]
  SVPWMG/3(Duty_C) -> duty_c/1
  SVPWMG/2(Duty_B) -> duty_b/1
  SVPWMG/1(Duty_A) -> duty_a/1
  [etheta] -> Park Transform/3
  ib/1 -> [ib], Clack/2(ib)
  ic/1 -> [ic], Clack/3(ic)
  ia/1 -> [ia], Clack/1(ia)
  iq_ref/1 -> [Iq_ref]
  [id] -> Id/2(id)
  [id] -> Iq/2(id)
  [iq] -> Id/3(iq)
  [iq] -> Iq/3(iq)
  Park Transform/1 -> [id], obs_id/1  "obs_id"
  Park Transform/2 -> obs_iq/1, [iq]  "obs_iq"
  [we] -> Id/4(we)
  [we] -> Iq/4(we)
  Inverse Park Transform/2 -> DeadTime_Compensation/2(Vbeta)
  DeadTime_Compensation/1(Valpha_comp) -> SVPWMG/1(Valpha)
  DeadTime_Compensation/2(Vbeta_comp) -> SVPWMG/2(Vbeta)
  Inverse Park Transform/1 -> DeadTime_Compensation/1(Valpha)
  [ia] -> DeadTime_Compensation/3(ia)
  [ib] -> DeadTime_Compensation/4(ib)
  [ic] -> DeadTime_Compensation/5(ic)
  [Id_Ref] -> DPCC_Current_Controller/1(id_ref_next)
  [Iq_ref] -> DPCC_Current_Controller/2(iq_ref_next)
  [id] -> DPCC_Current_Controller/3(id_meas)
  [iq] -> DPCC_Current_Controller/4(iq_meas)
  [we] -> DPCC_Current_Controller/5(we)
  [ud_raw] -> select_ud_current_mode/3
  [uq_raw] -> select_uq_current_mode/3
  DPCC_Current_Controller/1(ud_dpcc) -> [dpcc_ud]
  DPCC_Current_Controller/2(uq_dpcc) -> [dpcc_uq]
  [dpcc_ud] -> select_ud_current_mode/1
  [dpcc_uq] -> select_uq_current_mode/1
  select_ud_current_mode/1 -> [selected_ud_raw]
  [selected_ud_raw] -> dq_voltage_limiter/1(ud_raw)
  select_uq_current_mode/1 -> [selected_uq_raw]
  [selected_uq_raw] -> Switch2/3
  Current_Control_Mode/1 -> select_ud_current_mode/2, [mode]
  Current_Control_Mode1/1 -> select_uq_current_mode/2
  Close_Loop_EN/1 -> DPCC_Current_Controller/6(Close_Loop_EN)
  Angle_Init_EN/1 -> DPCC_Current_Controller/7(Angle_Init_EN)
  [mode] -> DPCC_Current_Controller/8(Current_Control_Mode)
  [ud_lim] -> DPCC_Current_Controller/9(ud_lim)
  [uq_lim] -> DPCC_Current_Controller/10(uq_lim)
  [ud_raw] -> DPCC_Current_Controller/11(ud_pi)
  [uq_raw] -> DPCC_Current_Controller/12(uq_pi)
  Init_Done/1 -> DPCC_Current_Controller/13(Init_Done)
  fault_latch/1 -> DPCC_Current_Controller/14(fault_latch)
  [ud_lim] -> vd_cmd/1, Inverse Park Transform/1  "ud_lim"
  [uq_lim] -> vq_cmd/1, Inverse Park Transform/2  "uq_lim"

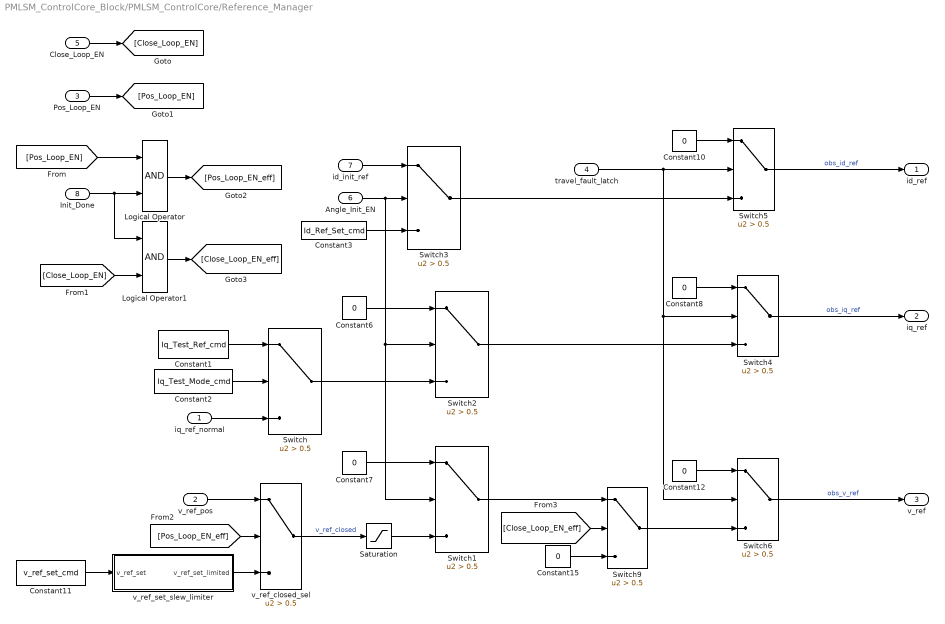
== system PMLSM_ControlCore_Block/PMLSM_ControlCore/Reference_Manager ==
  iq_ref_normal : Inport
  v_ref_pos : Inport  Port=2
  Pos_Loop_EN : Inport  Port=3
  travel_fault_latch : Inport  Port=4
  Close_Loop_EN : Inport  Port=5
  Angle_Init_EN : Inport  Port=6
  id_init_ref : Inport  Port=7
  Init_Done : Inport  Port=8
  Constant1 : DataStoreRead  DataStoreName=Iq_Test_Ref_cmd  IndexOptions=Index vector (dialog)  Indices=1  OutputSizes=1
  Constant{6..8,10,12,15} (6 alike) : Constant  Value=0
  Constant11 : DataStoreRead  DataStoreName=v_ref_set_cmd  IndexOptions=Index vector (dialog)  Indices=1  OutputSizes=1
  Constant2 : DataStoreRead  DataStoreName=Iq_Test_Mode_cmd  IndexOptions=Index vector (dialog)  Indices=1  OutputSizes=1
  Constant3 : DataStoreRead  DataStoreName=Id_Ref_Set_cmd  IndexOptions=Index vector (dialog)  Indices=1  OutputSizes=1
  Logical Operator : Logic  AllPortsSameDT=off  OutDataTypeStr=boolean
  Logical Operator1 : Logic  AllPortsSameDT=off  OutDataTypeStr=boolean
  Saturation : Saturate  UpperLimit=v_ref_max  LowerLimit=-v_ref_max
  Switch{,1..6,9} (8 alike) : Switch  Criteria=u2 > Threshold  Threshold=0.5  SaturateOnIntegerOverflow=off  InputSameDT=off
  v_ref_closed_sel : Switch  Criteria=u2 > Threshold  Threshold=0.5  SaturateOnIntegerOverflow=off  InputSameDT=off
  v_ref_set_slew_limiter : Subsystem
  id_ref : Outport
  iq_ref : Outport  Port=2
  v_ref : Outport  Port=3
  wires:
  [Pos_Loop_EN_eff] -> v_ref_closed_sel/2
  Logical Operator1/1 -> [Close_Loop_EN_eff]
  [Close_Loop_EN] -> Logical Operator1/2
  Logical Operator/1 -> [Pos_Loop_EN_eff]
  Init_Done/1 -> Logical Operator/2, Logical Operator1/1
  [Pos_Loop_EN] -> Logical Operator/1
  Pos_Loop_EN/1 -> [Pos_Loop_EN]
  Switch1/1 -> Switch9/1
  Switch9/1 -> Switch6/3
  [Close_Loop_EN_eff] -> Switch9/2
  Constant15/1 -> Switch9/3
  Switch6/1 -> v_ref/1  "obs_v_ref"
  Switch3/1 -> Switch5/3
  id_init_ref/1 -> Switch3/1
  Angle_Init_EN/1 -> Switch1/2, Switch2/2, Switch3/2
  Switch4/1 -> iq_ref/1  "obs_iq_ref"
  Switch5/1 -> id_ref/1  "obs_id_ref"
  Close_Loop_EN/1 -> [Close_Loop_EN]
  Saturation/1 -> Switch1/3
  Constant12/1 -> Switch6/1
  travel_fault_latch/1 -> Switch6/2, Switch4/2, Switch5/2
  Constant10/1 -> Switch5/1
  Constant8/1 -> Switch4/1
  Switch2/1 -> Switch4/3
  Switch/1 -> Switch2/3
  Constant6/1 -> Switch2/1
  Constant7/1 -> Switch1/1
  v_ref_closed_sel/1 -> Saturation/1  "v_ref_closed"
  v_ref_set_slew_limiter/1(v_ref_set_limited) -> v_ref_closed_sel/3
  v_ref_pos/1 -> v_ref_closed_sel/1
  iq_ref_normal/1 -> Switch/3
  Constant11/1 -> v_ref_set_slew_limiter/1(v_ref_set)
  Constant2/1 -> Switch/2
  Constant1/1 -> Switch/1
  Constant3/1 -> Switch3/3

== system PMLSM_ControlCore_Block/PMLSM_ControlCore/Scheduler_10k_1k_100 ==
  note: speed 计数链(/10)
  note: position 计数链(/100)
  note: 串口计数链(/10)
  Add1 : Sum
  Add2 : Sum
  Add3 : Sum
  Constant1 : Constant
  Constant2 : Constant  Value=0
  Constant3 : Constant
  Constant4 : Constant  Value=0
  Constant5 : Constant
  Constant6 : Constant  Value=0
  Logical Operator : Logic  AllPortsSameDT=off  OutDataTypeStr=boolean
  UART_cnt_next_sel : Switch  Criteria=u2 > Threshold  Threshold=0.5  SaturateOnIntegerOverflow=off  InputSameDT=off
  UART_cnt_z : UnitDelay  SampleTime=-1
  UART_tc : simulink/Logic and Bit Operations/Compare To Constant  relop=>=  const=10  OutDataTypeStr=boolean
  pos_cnt_hold_sel : Switch  Criteria=u2 > Threshold  Threshold=0.5  SaturateOnIntegerOverflow=off  InputSameDT=off
  pos_cnt_update_sel : Switch  Criteria=u2 > Threshold  Threshold=0.5  SaturateOnIntegerOverflow=off  InputSameDT=off
  pos_cnt_z : UnitDelay  SampleTime=-1
  pos_tc : simulink/Logic and Bit Operations/Compare To Constant  relop=>=  const=10  OutDataTypeStr=boolean
  spd_cnt_next_sel : Switch  Criteria=u2 > Threshold  Threshold=0.5  SaturateOnIntegerOverflow=off  InputSameDT=off
  spd_cnt_z : UnitDelay  SampleTime=-1
  spd_tc : simulink/Logic and Bit Operations/Compare To Constant  relop=>=  const=10  OutDataTypeStr=boolean
  UART_tick : Outport
  speed_tick : Outport  Port=2
  pos_tick : Outport  Port=3
  wires:
  Constant5/1 -> Add3/2
  UART_cnt_z/1 -> Add3/1
  Add3/1 -> UART_tc/1, UART_cnt_next_sel/3  "UART_cnt_inc"
  UART_cnt_next_sel/1 -> UART_cnt_z/1
  UART_tc/1 -> UART_cnt_next_sel/2, UART_tick/1
  Constant6/1 -> UART_cnt_next_sel/1
  Logical Operator/1 -> pos_tick/1
  pos_cnt_hold_sel/1 -> pos_cnt_z/1
  pos_cnt_update_sel/1 -> pos_cnt_hold_sel/1  "pos_cnt_update_candidate"
  Constant4/1 -> pos_cnt_update_sel/1
  pos_tc/1 -> pos_cnt_update_sel/2, Logical Operator/2
  Add2/1 -> pos_tc/1, pos_cnt_update_sel/3  "pos_cnt_inc"
  Constant3/1 -> Add2/2
  pos_cnt_z/1 -> pos_cnt_hold_sel/3, Add2/1
  Add1/1 -> spd_tc/1, spd_cnt_next_sel/3  "spd_cnt_inc"
  spd_cnt_next_sel/1 -> spd_cnt_z/1
  Constant2/1 -> spd_cnt_next_sel/1
  Constant1/1 -> Add1/2
  spd_tc/1 -> spd_cnt_next_sel/2, pos_cnt_hold_sel/2, Logical Operator/1, speed_tick/1
  spd_cnt_z/1 -> Add1/1

== system PMLSM_ControlCore_Block/PMLSM_ControlCore/Triggered_Position_loop ==
  x_ref_mm : Inport
  x_mm : Inport  Port=2
  pos_pi_reset : Inport  Port=3
  v_ff_pos : Inport  Port=4
  Trigger : TriggerPort  VariantControl=(inherit)
  Dead Zone : DeadZone  LowerValue=-Pos_deadband  UpperValue=+Pos_deadband
  Gain : Gain  Gain=Kp_pos
  Saturation : Saturate  UpperLimit=V_pos_max_mmps  LowerLimit=-V_pos_max_mmps
  Sum : Sum  Inputs=|+-
  Sum1 : Sum  Inputs=|++
  Terminator : Terminator
  v_ref_pos : Outport
  wires:
  Saturation/1 -> v_ref_pos/1  "obs_v_ref_pos"
  pos_pi_reset/1 -> Terminator/1
  Sum1/1 -> Saturation/1
  v_ff_pos/1 -> Sum1/2
  Gain/1 -> Sum1/1
  Dead Zone/1 -> Gain/1
  Sum/1 -> Dead Zone/1  "e_pos"
  x_mm/1 -> Sum/2
  x_ref_mm/1 -> Sum/1

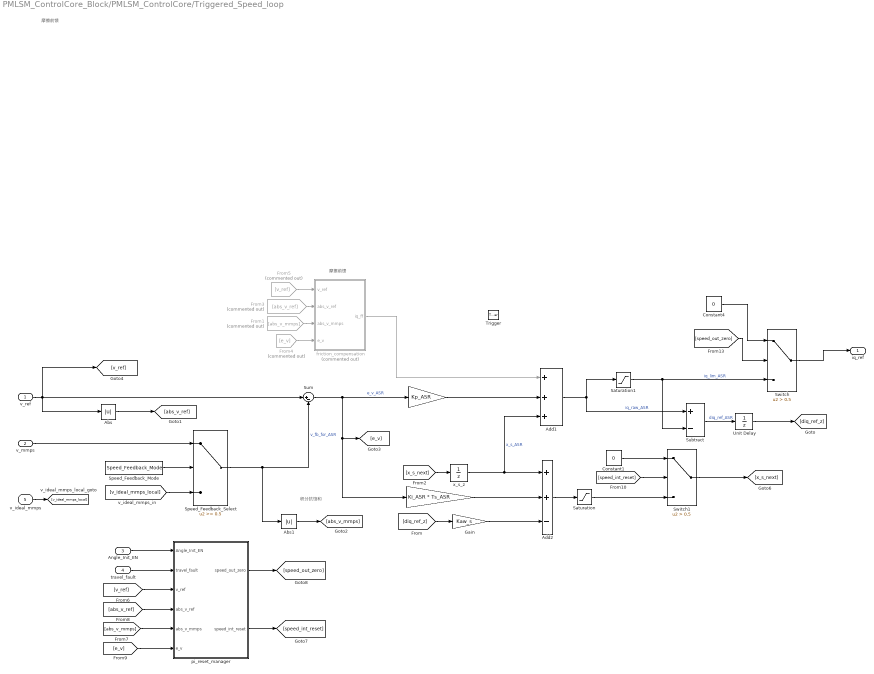
== system PMLSM_ControlCore_Block/PMLSM_ControlCore/Triggered_Speed_loop ==
  note: 摩擦前馈
  note: 积分抗饱和
  note: 摩擦前馈
  v_ref : Inport
  v_mmps : Inport  Port=2
  Angle_Init_EN : Inport  Port=3
  travel_fault : Inport  Port=4
  v_ideal_mmps : Inport  Port=5
  Trigger : TriggerPort  VariantControl=(inherit)
  " " : Gain  Gain=Ki_ASR * Ts_ASR
  "  " : Gain  Gain=Kp_ASR
  Abs : Abs  SaturateOnIntegerOverflow=off
  Abs1 : Abs  SaturateOnIntegerOverflow=off
  Add1 : Sum  Inputs=+++
  Add2 : Sum  Inputs=++-
  Constant1 : Constant  Value=0
  Constant4 : Constant  Value=0
  From1 : From  Commented=on  GotoTag=abs_v_mmps
  From3 : From  Commented=on  GotoTag=abs_v_ref
  From4 : From  Commented=on  GotoTag=e_v
  From5 : From  Commented=on  GotoTag=v_ref
  Gain : Gain  Gain=Kaw_s
  Saturation : Saturate  UpperLimit=Iq_int_limit  LowerLimit=-Iq_int_limit
  Saturation1 : Saturate  UpperLimit=Speed_loop_Iq_Limit  LowerLimit=-Speed_loop_Iq_Limit
  Speed_Feedback_Mode : Constant  Value=Speed_Feedback_Mode
  Speed_Feedback_Select : Switch  Threshold=0.5  SaturateOnIntegerOverflow=off  InputSameDT=off
  Subtract : Sum  Inputs=+-
  Sum : Sum  Inputs=|+-
  Switch : Switch  Criteria=u2 > Threshold  Threshold=0.5  SaturateOnIntegerOverflow=off  InputSameDT=off
  Switch1 : Switch  Criteria=u2 > Threshold  Threshold=0.5  SaturateOnIntegerOverflow=off  InputSameDT=off
  Unit Delay : UnitDelay  SampleTime=-1
  friction_compensation : Subsystem  Commented=on
  pi_reset_manager : Subsystem
  x_s_z : UnitDelay  SampleTime=-1
  iq_ref : Outport
  wires:
  Saturation/1 -> Switch1/3
  Switch1/1 -> [x_s_next]
  [speed_int_reset] -> Switch1/2
  pi_reset_manager/1(speed_out_zero) -> [speed_out_zero]
  pi_reset_manager/2(speed_int_reset) -> [speed_int_reset]
  [speed_out_zero] -> Switch/2
  [e_v] -> pi_reset_manager/6(e_v)
  [abs_v_ref] -> pi_reset_manager/4(abs_v_ref)
  [abs_v_mmps] -> pi_reset_manager/5(abs_v_mmps)
  [v_ref] -> pi_reset_manager/3(v_ref)
  From5/1 -> friction_compensation/1(v_ref)
  travel_fault/1 -> pi_reset_manager/2(travel_fault)
  Angle_Init_EN/1 -> pi_reset_manager/1(Angle_Init_EN)
  Abs1/1 -> [abs_v_mmps]
  Abs/1 -> [abs_v_ref]
  From3/1 -> friction_compensation/2(abs_v_ref)
  From1/1 -> friction_compensation/3(abs_v_mmps)
  From4/1 -> friction_compensation/4(e_v)
  x_s_z/1 -> Add2/1, Add1/3  "x_s_ASR"
  friction_compensation/1(iq_ff) -> Add1/1
  "  "/1 -> Add1/2
  Constant4/1 -> Switch/1
  Switch/1 -> iq_ref/1
  Constant1/1 -> Switch1/1
  [diq_ref_z] -> Gain/1
  Unit Delay/1 -> [diq_ref_z]
  Subtract/1 -> Unit Delay/1  "diq_ref_ASR"
  " "/1 -> Add2/2
  Gain/1 -> Add2/3
  Add2/1 -> Saturation/1
  [x_s_next] -> x_s_z/1
  Saturation1/1 -> Subtract/2, Switch/3  "iq_lim_ASR"
  v_ref/1 -> [v_ref], Abs/1, Sum/1
  Add1/1 -> Saturation1/1, Subtract/1  "iq_raw_ASR"
  Sum/1 -> " "/1, [e_v], "  "/1  "e_v_ASR"
  v_ideal_mmps/1 -> [v_ideal_mmps_local]
  v_mmps/1 -> Speed_Feedback_Select/1
  Speed_Feedback_Mode/1 -> Speed_Feedback_Select/2
  [v_ideal_mmps_local] -> Speed_Feedback_Select/3
  Speed_Feedback_Select/1 -> Sum/2, Abs1/1  "v_fb_for_ASR"

== system PMLSM_ControlCore_Block/PMLSM_ControlCore/Caculate_measurement/IIR Filter ==
  In1 : Inport
  Reset : ResetPort  DisableCoverage=on
  IIR Filter : mcbcontrolslib/IIR Filter  VariantControl=Low Pass Filter  VariantSelect=Low-pass  FilterConstantInputType=Specify via dialog  Filter_constant=0.1  InitialOutput=Specify via dialog  InitialOutputValue=0  ExternalReset=none  advancedSettings=on  Ts=100e-6  cutOff_freq=176.8388
  Out1 : Outport
  wires:
  IIR Filter/1 -> Out1/1
  In1/1 -> IIR Filter/1

== system PMLSM_ControlCore_Block/PMLSM_ControlCore/FOC_Algorithm/Clack ==
  note: alpha=(A-0.5*(B+C))*2/3
      | Beta=sqrt(3)/2*(B-C)*2/3
  ia : Inport
  ib : Inport  Port=2
  ic : Inport  Port=3
  Add : Sum  Inputs=+--
  Add1 : Sum  Inputs=+-
  Gain : Gain  Gain=0.5
  Gain1 : Gain  Gain=0.5
  Gain2 : Gain  Gain=2/3
  Gain3 : Gain  Gain=1/sqrt(3)
  ialpha : Outport
  ibeta : Outport  Port=2
  wires:
  Gain/1 -> Add/2
  Gain2/1 -> ialpha/1  "ialf"
  Add/1 -> Gain2/1
  Gain3/1 -> ibeta/1  "ibeta"
  ic/1 -> Gain1/1, Add1/2
  Add1/1 -> Gain3/1
  ib/1 -> Gain/1, Add1/1
  ia/1 -> Add/1
  Gain1/1 -> Add/3

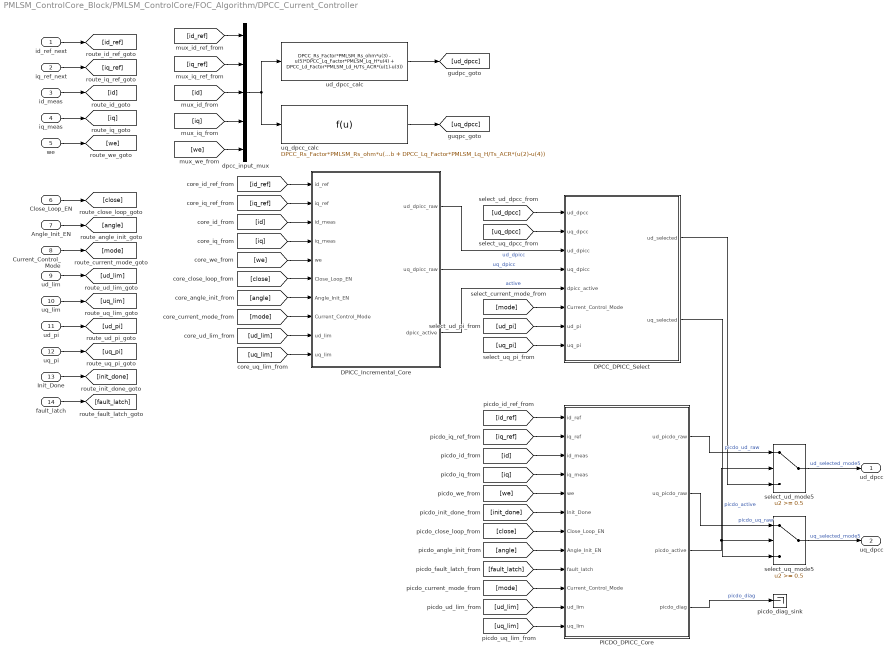
== system PMLSM_ControlCore_Block/PMLSM_ControlCore/FOC_Algorithm/DPCC_Current_Controller ==
  id_ref_next : Inport
  iq_ref_next : Inport  Port=2
  id_meas : Inport  Port=3
  iq_meas : Inport  Port=4
  we : Inport  Port=5
  Close_Loop_EN : Inport  Port=6
  Angle_Init_EN : Inport  Port=7
  Current_Control_Mode : Inport  Port=8
  ud_lim : Inport  Port=9
  uq_lim : Inport  Port=10
  ud_pi : Inport  Port=11
  uq_pi : Inport  Port=12
  Init_Done : Inport  Port=13
  fault_latch : Inport  Port=14
  DPCC_DPICC_Select : Subsystem
  DPICC_Incremental_Core : Subsystem
  PICDO_DPICC_Core : Subsystem
  dpcc_input_mux : Mux  Inputs=5
  picdo_diag_sink : Terminator
  select_ud_mode5 : Switch  Threshold=0.5
  select_uq_mode5 : Switch  Threshold=0.5
  ud_dpcc_calc : Fcn  Expr=DPCC_Rs_Factor*PMLSM_Rs_ohm*u(3) - u(5)*DPCC_Lq_Factor*PMLSM_Lq_H*u(4) + DPCC_Ld_Factor*PMLSM_Ld_H/Ts_ACR*(u(1)-u(3))
  uq_dpcc_calc : Fcn  Expr=DPCC_Rs_Factor*PMLSM_Rs_ohm*u(4) + u(5)*DPCC_Ld_Factor*PMLSM_Ld_H*u(3) + u(5)*DPCC_Psi_Factor*PMLSM_psi_f_Wb + DPCC_Lq_Factor*PMLSM_Lq_H/Ts_ACR*(u(2)-u(4))
  ud_dpcc : Outport
  uq_dpcc : Outport  Port=2
  wires:
  dpcc_input_mux/1 -> uq_dpcc_calc/1, ud_dpcc_calc/1
  id_ref_next/1 -> [id_ref]
  iq_ref_next/1 -> [iq_ref]
  id_meas/1 -> [id]
  iq_meas/1 -> [iq]
  we/1 -> [we]
  Close_Loop_EN/1 -> [close]
  Angle_Init_EN/1 -> [angle]
  Current_Control_Mode/1 -> [mode]
  ud_lim/1 -> [ud_lim]
  uq_lim/1 -> [uq_lim]
  ud_pi/1 -> [ud_pi]
  uq_pi/1 -> [uq_pi]
  [id_ref] -> dpcc_input_mux/1
  [iq_ref] -> dpcc_input_mux/2
  [id] -> dpcc_input_mux/3
  [iq] -> dpcc_input_mux/4
  [we] -> dpcc_input_mux/5
  [id_ref] -> DPICC_Incremental_Core/1(id_ref)
  [iq_ref] -> DPICC_Incremental_Core/2(iq_ref)
  [id] -> DPICC_Incremental_Core/3(id_meas)
  [iq] -> DPICC_Incremental_Core/4(iq_meas)
  [we] -> DPICC_Incremental_Core/5(we)
  [close] -> DPICC_Incremental_Core/6(Close_Loop_EN)
  [angle] -> DPICC_Incremental_Core/7(Angle_Init_EN)
  [mode] -> DPICC_Incremental_Core/8(Current_Control_Mode)
  [ud_lim] -> DPICC_Incremental_Core/9(ud_lim)
  [uq_lim] -> DPICC_Incremental_Core/10(uq_lim)
  [ud_dpcc] -> DPCC_DPICC_Select/1(ud_dpcc)
  [uq_dpcc] -> DPCC_DPICC_Select/2(uq_dpcc)
  [mode] -> DPCC_DPICC_Select/6(Current_Control_Mode)
  [ud_pi] -> DPCC_DPICC_Select/7(ud_pi)
  [uq_pi] -> DPCC_DPICC_Select/8(uq_pi)
  ud_dpcc_calc/1 -> [ud_dpcc]
  uq_dpcc_calc/1 -> [uq_dpcc]
  DPICC_Incremental_Core/1(ud_dpicc_raw) -> DPCC_DPICC_Select/3(ud_dpicc)  "ud_dpicc"
  DPICC_Incremental_Core/2(uq_dpicc_raw) -> DPCC_DPICC_Select/4(uq_dpicc)  "uq_dpicc"
  DPICC_Incremental_Core/3(dpicc_active) -> DPCC_DPICC_Select/5(dpicc_active)  "active"
  DPCC_DPICC_Select/1(ud_selected) -> select_ud_mode5/3
  DPCC_DPICC_Select/2(uq_selected) -> select_uq_mode5/3
  select_ud_mode5/1 -> ud_dpcc/1  "ud_selected_mode5"
  select_uq_mode5/1 -> uq_dpcc/1  "uq_selected_mode5"
  PICDO_DPICC_Core/1(ud_picdo_raw) -> select_ud_mode5/1  "picdo_ud_raw"
  PICDO_DPICC_Core/2(uq_picdo_raw) -> select_uq_mode5/1  "picdo_uq_raw"
  PICDO_DPICC_Core/3(picdo_active) -> select_uq_mode5/2, select_ud_mode5/2  "picdo_active"
  PICDO_DPICC_Core/4(picdo_diag) -> picdo_diag_sink/1  "picdo_diag"
  Init_Done/1 -> [init_done]
  fault_latch/1 -> [fault_latch]
  [id_ref] -> PICDO_DPICC_Core/1(id_ref)
  [iq_ref] -> PICDO_DPICC_Core/2(iq_ref)
  [id] -> PICDO_DPICC_Core/3(id_meas)
  [iq] -> PICDO_DPICC_Core/4(iq_meas)
  [we] -> PICDO_DPICC_Core/5(we)
  [init_done] -> PICDO_DPICC_Core/6(Init_Done)
  [close] -> PICDO_DPICC_Core/7(Close_Loop_EN)
  [angle] -> PICDO_DPICC_Core/8(Angle_Init_EN)
  [fault_latch] -> PICDO_DPICC_Core/9(fault_latch)
  [mode] -> PICDO_DPICC_Core/10(Current_Control_Mode)
  [ud_lim] -> PICDO_DPICC_Core/11(ud_lim)
  [uq_lim] -> PICDO_DPICC_Core/12(uq_lim)

== system PMLSM_ControlCore_Block/PMLSM_ControlCore/FOC_Algorithm/DeadTime_Compensation ==
  Valpha : Inport
  Vbeta : Inport  Port=2
  ia : Inport  Port=3
  ib : Inport  Port=4
  ic : Inport  Port=5
  add_valpha_comp : Sum
  add_vbeta_comp : Sum
  phase_comp_mux : Mux  Inputs=3
  phase_to_valpha_comp : Fcn  Expr=(2/3)*(u[1]-0.5*u[2]-0.5*u[3])
  phase_to_vbeta_comp : Fcn  Expr=0.577350269189626*(u[2]-u[3])
  sign_a : Fcn  Expr=(u > PMLSM_deadtime_current_eps_A) - (u < -PMLSM_deadtime_current_eps_A)
  sign_b : Fcn  Expr=(u > PMLSM_deadtime_current_eps_A) - (u < -PMLSM_deadtime_current_eps_A)
  sign_c : Fcn  Expr=(u > PMLSM_deadtime_current_eps_A) - (u < -PMLSM_deadtime_current_eps_A)
  vcomp_a : Gain  Gain=Udc*PMLSM_deadtime_ratio*DeadTime_Comp_Enable
  vcomp_b : Gain  Gain=Udc*PMLSM_deadtime_ratio*DeadTime_Comp_Enable
  vcomp_c : Gain  Gain=Udc*PMLSM_deadtime_ratio*DeadTime_Comp_Enable
  Valpha_comp : Outport
  Vbeta_comp : Outport  Port=2
  wires:
  ia/1 -> sign_a/1
  sign_a/1 -> vcomp_a/1
  vcomp_a/1 -> phase_comp_mux/1
  ib/1 -> sign_b/1
  sign_b/1 -> vcomp_b/1
  vcomp_b/1 -> phase_comp_mux/2
  ic/1 -> sign_c/1
  sign_c/1 -> vcomp_c/1
  vcomp_c/1 -> phase_comp_mux/3
  Valpha/1 -> add_valpha_comp/1
  Vbeta/1 -> add_vbeta_comp/1
  phase_to_valpha_comp/1 -> add_valpha_comp/2
  phase_to_vbeta_comp/1 -> add_vbeta_comp/2
  add_valpha_comp/1 -> Valpha_comp/1
  add_vbeta_comp/1 -> Vbeta_comp/1
  phase_comp_mux/1 -> phase_to_valpha_comp/1, phase_to_vbeta_comp/1

== system PMLSM_ControlCore_Block/PMLSM_ControlCore/FOC_Algorithm/Id ==
  note: 起到使能时初始化一下的作用
  id_ref : Inport
  id : Inport  Port=2
  iq : Inport  Port=3
  we : Inport  Port=4
  du_d_z : Inport  Port=5
  " " : Gain  Gain=Ki_ACR*Ts_ACR
  "  " : Gain  Gain=Kp_ACR
  Add1 : Sum
  Add2 : Sum  Inputs=++-
  Constant : DataStoreRead  DataStoreName=PI_Reset_EN_cmd  IndexOptions=Index vector (dialog)  Indices=1  OutputSizes=1
  Constant1 : Constant  Value=PMLSM_Lq_H
  Constant2 : Constant  Value=0
  Constant3 : Constant  Value=0
  Gain : Gain  Gain=Kaw_d
  Product : Product
  Product1 : Product
  Sum : Sum  Inputs=|+-
  Sum1 : Sum  Inputs=|+-
  Switch : Switch  Criteria=u2 > Threshold  Threshold=0.5  SaturateOnIntegerOverflow=off  InputSameDT=off
  Switch1 : Switch  Criteria=u2 > Threshold  Threshold=0.5  SaturateOnIntegerOverflow=off  InputSameDT=off
  x_d_z : UnitDelay  SampleTime=-1
  ud_raw : Outport
  wires:
  Switch1/1 -> [x_d_next]
  Constant3/1 -> Switch1/1
  " "/1 -> Add2/2  "KiTs_q * e_d"
  [du_d_z] -> Gain/1
  Gain/1 -> Add2/3  "u_d,aw"
  Add2/1 -> Switch1/3  "x_d_next"
  [x_d_next] -> x_d_z/1
  x_d_z/1 -> Add2/1, Add1/2
  du_d_z/1 -> [du_d_z]
  Switch/1 -> ud_raw/1  "obs_ud_raw"
  Sum1/1 -> Switch/3
  Constant2/1 -> Switch/1
  "  "/1 -> Add1/1
  Constant/1 -> Switch/2, Switch1/2
  Constant1/1 -> Product/2
  Add1/1 -> Sum1/1
  Product/1 -> Product1/1
  we/1 -> Product1/2
  Product1/1 -> Sum1/2  "解耦项"
  Sum/1 -> "  "/1, " "/1
  id/1 -> Sum/2
  id_ref/1 -> Sum/1
  iq/1 -> Product/1

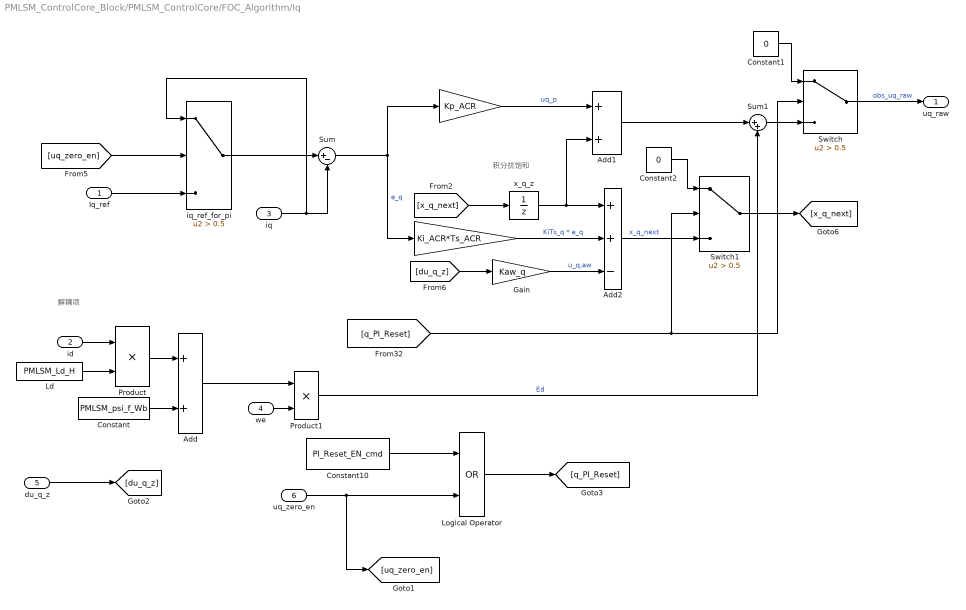
== system PMLSM_ControlCore_Block/PMLSM_ControlCore/FOC_Algorithm/Iq ==
  note: 积分抗饱和
  note: 解耦项
  Iq_ref : Inport
  id : Inport  Port=2
  iq : Inport  Port=3
  we : Inport  Port=4
  du_q_z : Inport  Port=5
  uq_zero_en : Inport  Port=6
  " " : Gain  Gain=Ki_ACR*Ts_ACR
  "  " : Gain  Gain=Kp_ACR
  Add : Sum
  Add1 : Sum
  Add2 : Sum  Inputs=++-
  Constant : Constant  Value=PMLSM_psi_f_Wb
  Constant1 : Constant  Value=0
  Constant10 : DataStoreRead  DataStoreName=PI_Reset_EN_cmd  IndexOptions=Index vector (dialog)  Indices=1  OutputSizes=1
  Constant2 : Constant  Value=0
  Gain : Gain  Gain=Kaw_q
  Ld : Constant  Value=PMLSM_Ld_H
  Logical Operator : Logic  Operator=OR  AllPortsSameDT=off  OutDataTypeStr=boolean
  Product : Product
  Product1 : Product
  Sum : Sum  Inputs=|+-
  Sum1 : Sum  Inputs=|++
  Switch : Switch  Criteria=u2 > Threshold  Threshold=0.5  SaturateOnIntegerOverflow=off  InputSameDT=off
  Switch1 : Switch  Criteria=u2 > Threshold  Threshold=0.5  SaturateOnIntegerOverflow=off  InputSameDT=off
  iq_ref_for_pi : Switch  Criteria=u2 > Threshold  Threshold=0.5  SaturateOnIntegerOverflow=off  InputSameDT=off
  x_q_z : UnitDelay  SampleTime=-1
  uq_raw : Outport
  wires:
  Logical Operator/1 -> [q_PI_Reset]
  uq_zero_en/1 -> Logical Operator/2, [uq_zero_en]
  [x_q_next] -> x_q_z/1
  Switch1/1 -> [x_q_next]
  Add2/1 -> Switch1/3  "x_q_next"
  Constant2/1 -> Switch1/1
  x_q_z/1 -> Add2/1, Add1/2
  " "/1 -> Add2/2  "KiTs_q * e_q"
  Gain/1 -> Add2/3  "u_q,aw"
  [du_q_z] -> Gain/1
  iq_ref_for_pi/1 -> Sum/1
  Iq_ref/1 -> iq_ref_for_pi/3
  [uq_zero_en] -> iq_ref_for_pi/2
  du_q_z/1 -> [du_q_z]
  [q_PI_Reset] -> Switch1/2, Switch/2
  Sum1/1 -> Switch/3
  Switch/1 -> uq_raw/1  "obs_uq_raw"
  Constant1/1 -> Switch/1
  "  "/1 -> Add1/1  "uq_p"
  Sum/1 -> " "/1, "  "/1  "e_q"
  Add/1 -> Product1/1
  Constant/1 -> Add/2
  Product/1 -> Add/1
  Ld/1 -> Product/2
  id/1 -> Product/1
  iq/1 -> Sum/2, iq_ref_for_pi/1
  Add1/1 -> Sum1/1
  we/1 -> Product1/2
  Product1/1 -> Sum1/2  "Ed"
  Constant10/1 -> Logical Operator/1

== system PMLSM_ControlCore_Block/PMLSM_ControlCore/FOC_Algorithm/SVPWMG ==
  Valpha : Inport
  Vbeta : Inport  Port=2
  Duty Calculate : Subsystem  TreatAsAtomicUnit=on  RTWFcnName=Duty_Caculate_Fun
      settings: RTWFcnNameOpts=User specified
  Sector Caculate : Subsystem  TreatAsAtomicUnit=on  RTWFcnName=Sector_Caculate_Fun
      settings: RTWFcnNameOpts=User specified
  T1T2 Calculate : Subsystem  TreatAsAtomicUnit=on  RTWFcnName=T1T2Caculate_Fun
      settings: RTWFcnNameOpts=User specified
  Udc : Constant  Value=Udc
  XYZ Calculate : Subsystem  TreatAsAtomicUnit=on  RTWFcnName=XYZ_Caculate_Fun
      settings: RTWFcnNameOpts=User specified
  Duty_A : Outport
  Duty_B : Outport  Port=2
  Duty_C : Outport  Port=3
  "N " : Outport  Port=4
  wires:
  Duty Calculate/3(Duty_W) -> Duty_C/1
  Duty Calculate/2(Duty_V) -> Duty_B/1
  Duty Calculate/1(Duty_U) -> Duty_A/1
  XYZ Calculate/3(Z) -> T1T2 Calculate/4(Z)
  XYZ Calculate/2(Y) -> T1T2 Calculate/3(Y)
  XYZ Calculate/1(X) -> T1T2 Calculate/2(X)
  Udc/1 -> XYZ Calculate/3(Udc)
  Sector Caculate/1("N ") -> T1T2 Calculate/1(N), Duty Calculate/1(N), "N "/1
  T1T2 Calculate/2(T2) -> Duty Calculate/3(T2)
  Valpha/1 -> XYZ Calculate/1(Ualpha), Sector Caculate/1(Ualpha)
  T1T2 Calculate/1(T1) -> Duty Calculate/2(T1)
  Vbeta/1 -> XYZ Calculate/2(Ubeta), Sector Caculate/2(Ubeta)
